simulink model "model"  (R2014b)
settings: Solver=ode4  StartTime=0.0  StopTime=10  FixedStep=0.01  RelTol=1e-3
values from neighbouring files (symbols this model uses):
  alp_trim = [0.0586239258484  0.0724982110928  0.103723100468; 0.0422368784565  0.0555720453493  0.0854543358165; 0.0309898683799  0.0444507527561  0.0743831948455]    [matlab.mat]    (also in plot_result.m = simOut.get('alp_trim')*r2d; plot_result_2.m = simOut.get('alp_trim')*r2d)
  dele_trim = [-0.00382132885472  -0.0381952981036  -0.0862584503139; 0.004502506619  -0.0421428537274  -0.104658611065; 0.0106660878134  -0.0496771115948  -0.12971922856]    [matlab.mat]
  delt_trim = [0.188785278717  0.195588305395  0.214097966619; 0.206526466279  0.211744859207  0.226730875318; 0.229775096744  0.233650878336  0.246767074549]    [matlab.mat]    (also in plot_result.m = simOut.get('delt_trim'); plot_result_2.m = simOut.get('delt_trim'))
undefined symbols (not defined in the file or in its folder): sigbuilder_block
libraries: aerolibconvert2 x9, LPVBlockLibrary x1, aerolibactuator x1
settings Model: Creator=jihoo  LastModifiedBy=Jihoon Lee

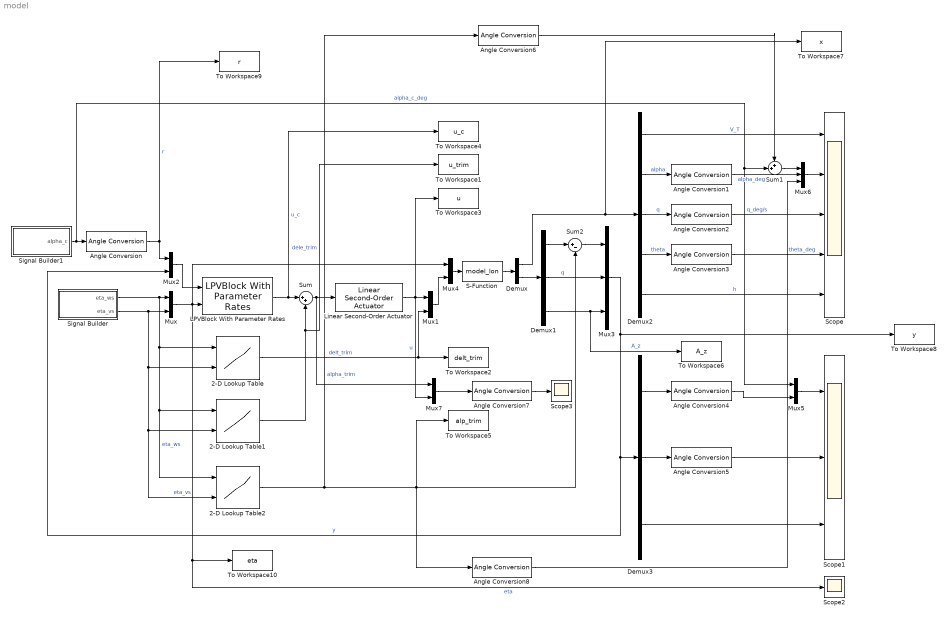
== system model ==
  2-D Lookup Table : Lookup_n-D  BreakpointsForDimension1=[0:0.5:1]  BreakpointsForDimension2=[0:0.5:1]  Table=delt_trim  InternalRulePriority=Speed  RndMeth=Simplest  InputSameDT=on
  2-D Lookup Table1 : Lookup_n-D  BreakpointsForDimension1=[0:0.5:1]  BreakpointsForDimension2=[0:0.5:1]  Table=dele_trim  InternalRulePriority=Speed  RndMeth=Simplest  InputSameDT=on
  2-D Lookup Table2 : Lookup_n-D  BreakpointsForDimension1=[0:0.5:1]  BreakpointsForDimension2=[0:0.5:1]  Table=alp_trim  InternalRulePriority=Speed  RndMeth=Simplest  InputSameDT=on
  Angle Conversion : aerolibconvert2/Angle Conversion  IU=deg  OU=rad
  Angle Conversion{1..8} (8 alike) : aerolibconvert2/Angle Conversion  IU=rad  OU=deg
  Demux : Demux  Outputs=[5 3]
  Demux1 : Demux  Outputs=[1 1 1]
  Demux2 : Demux  Outputs=5
  Demux3 : Demux  Outputs=3
  LPVBlock With Parameter Rates : LPVBlockLibrary/LPVBlock With Parameter Rates  sys=Knr  plist={'eta1';'eta2'}  x0=zeros(7,1)  ratetc={'eta1',0.5;'eta2',0.5}
  Linear Second-Order Actuator : aerolibactuator/Linear Second-Order Actuator  wn_fin=105  z_fin=0.6  fin_act_0=dele_trim(1,2)  fin_act_vel=0
  Mux : Mux  Inputs=2
  Mux1 : Mux  Inputs=2
  Mux2 : Mux  Inputs=[1 3]
  Mux3 : Mux  Inputs=[1 1 1]
  Mux4 : Mux  Inputs=[2 2]
  Mux5 : Mux  Inputs=2
  Mux6 : Mux  Inputs=[1 1 1]
  Mux7 : Mux  Inputs=[1 1]
  S-Function : S-Function  FunctionName=model_lon  EnableBusSupport=off
  Scope : Scope  NumInputPorts=5
      settings: YMin=16~2~-15~-10~294  YMax=24~5.5~10~15~308
  Scope1 : Scope  NumInputPorts=3
      settings: YMin=-5~-5~-5  YMax=5~5~5
  Scope2 : Scope
      settings: SaveName=ScopeData2
  Scope3 : Scope
      settings: ShowLegends=on  YMin=-8  YMax=1  SaveName=ScopeData3
  Signal Builder : Subsystem  Tag=STV Subsys  LoadFcn=sigbuilder_block('load',[0 -216 1861.5 1017 ]);  StartFcn=sigbuilder_block('start');  StopFcn=sigbuilder_block('stop');  ClipboardFcn=sigbuilder_block('clipboard');  mask(Sigbuilder block){}
      mask help: Simulink:masks:SigbuilderBlock_MD
      mask init:
      | if ~strcmp(get_param(bdroot(gcbh),'SimulationStatus'),'stopped') tuvar = sigbuilder_block('maskInit'); end
      settings: CopyFcn=sigbuilder_block('copy');  DeleteFcn=sigbuilder_block('delete');  ModelCloseFcn=sigbuilder_block('modelClose');  PreSaveFcn=sigbuilder_block('preSave');  PauseFcn=sigbuilder_block('pause');  ContinueFcn=sigbuilder_block('continue');  NameChangeFcn=sigbuilder_block('namechange');  OpenFcn=sigbuilder_block('open',[437.6 199.2 550.4 400 ]);  CloseFcn=sigbuilder_block('close');
      mask Display: plot(0, 0, 100, 100,[2, 2, 32, 32, 2], [68, 8, 8, 68, 68],[32, 2], [38, 38], [32, 19, 2],[53, 60, 44], [32, 17, 17, 2],[16, 16, 31, 31]);txt = getActiveGroup(gcbh);text(2, 100, txt,'verticalAlignment', 'top');
  Signal Builder1 : Subsystem  Tag=STV Subsys  LoadFcn=sigbuilder_block('load');  StartFcn=sigbuilder_block('start');  StopFcn=sigbuilder_block('stop');  ClipboardFcn=sigbuilder_block('clipboard');  mask(Sigbuilder block){}
      mask help: Simulink:masks:SigbuilderBlock_MD
      mask init:
      | if ~strcmp(get_param(bdroot(gcbh),'SimulationStatus'),'stopped') tuvar = sigbuilder_block('maskInit'); end
      settings: CopyFcn=sigbuilder_block('copy');  DeleteFcn=sigbuilder_block('delete');  ModelCloseFcn=sigbuilder_block('modelClose');  PreSaveFcn=sigbuilder_block('preSave');  PauseFcn=sigbuilder_block('pause');  ContinueFcn=sigbuilder_block('continue');  NameChangeFcn=sigbuilder_block('namechange');  OpenFcn=sigbuilder_block('open',[437.6 199.2 550.4 400 ]);  CloseFcn=sigbuilder_block('close');
      mask Display: plot(0, 0, 100, 100,[2, 2, 32, 32, 2], [68, 8, 8, 68, 68],[32, 2], [38, 38], [32, 19, 2],[53, 60, 44], [32, 17, 17, 2],[16, 16, 31, 31]);txt = getActiveGroup(gcbh);text(2, 100, txt,'verticalAlignment', 'top');
  Sum : Sum  Inputs=|++
  Sum1 : Sum  Inputs=++|
  Sum2 : Sum  Inputs=|+-
  To Workspace1 : ToWorkspace  VariableName=u_trim  SampleTime=-1
      settings: Save2DSignal=2-D array (concatenate along first dimension)
  To Workspace10 : ToWorkspace  VariableName=eta  SampleTime=-1
      settings: Save2DSignal=2-D array (concatenate along first dimension)
  To Workspace2 : ToWorkspace  VariableName=delt_trim  SampleTime=-1
      settings: Save2DSignal=2-D array (concatenate along first dimension)
  To Workspace3 : ToWorkspace  VariableName=u  SampleTime=-1
      settings: Save2DSignal=2-D array (concatenate along first dimension)
  To Workspace4 : ToWorkspace  VariableName=u_c  SampleTime=-1
      settings: Save2DSignal=2-D array (concatenate along first dimension)
  To Workspace5 : ToWorkspace  VariableName=alp_trim  SampleTime=-1
      settings: Save2DSignal=2-D array (concatenate along first dimension)
  To Workspace6 : ToWorkspace  VariableName=A_z  SampleTime=-1
      settings: Save2DSignal=2-D array (concatenate along first dimension)
  To Workspace7 : ToWorkspace  VariableName=x  SampleTime=-1
      settings: Save2DSignal=2-D array (concatenate along first dimension)
  To Workspace8 : ToWorkspace  VariableName=y  SampleTime=-1
      settings: Save2DSignal=2-D array (concatenate along first dimension)
  To Workspace9 : ToWorkspace  VariableName=r  SampleTime=-1
      settings: Save2DSignal=2-D array (concatenate along first dimension)
  wires:
  Signal Builder/1(eta_ws) -> 2-D Lookup Table2/1, 2-D Lookup Table1/1, 2-D Lookup Table/1, Mux/1  "eta_ws"
  Signal Builder/2(eta_vs) -> 2-D Lookup Table2/2, 2-D Lookup Table1/2, 2-D Lookup Table/2, Mux/2  "eta_vs"
  Mux/1 -> Mux4/1, To Workspace10/1, Scope2/1, LPVBlock With Parameter Rates/2  "eta"
  S-Function/1 -> Demux/1
  Mux2/1 -> LPVBlock With Parameter Rates/1
  LPVBlock With Parameter Rates/1 -> To Workspace4/1, Sum/1  "u_c"
  2-D Lookup Table/1 -> To Workspace2/1, Mux1/2  "delt_trim"
  2-D Lookup Table1/1 -> To Workspace1/1, Sum/2  "dele_trim"
  2-D Lookup Table2/1 -> Angle Conversion6/1, Angle Conversion8/1, To Workspace5/1, Sum2/2  "alpha_trim"
  Demux/2 -> Demux1/1
  Demux/1 -> To Workspace7/1, Demux2/1
  Demux1/1 -> Sum2/1
  Sum2/1 -> Mux3/1
  Demux1/2 -> Mux3/2  "q"
  Demux1/3 -> To Workspace6/1, Mux3/3  "A_z"
  Mux3/1 -> Demux3/1, Mux2/2, To Workspace8/1  "y"
  Angle Conversion/1 -> Mux2/1, To Workspace9/1  "r"
  Sum/1 -> Linear Second-Order Actuator/1, Mux7/1
  Linear Second-Order Actuator/1 -> Mux7/2, To Workspace3/1, Mux1/1  "u"
  Mux4/1 -> S-Function/1
  Mux1/1 -> Mux4/2
  Demux3/1 -> Angle Conversion4/1
  Demux3/2 -> Angle Conversion5/1
  Demux3/3 -> Scope1/3
  Demux2/1 -> Scope/1  "V_T"
  Demux2/2 -> Angle Conversion1/1  "alpha"
  Demux2/3 -> Angle Conversion2/1  "q"
  Demux2/4 -> Angle Conversion3/1  "theta"
  Demux2/5 -> Scope/5  "h"
  Angle Conversion2/1 -> Scope/3  "q_deg/s"
  Angle Conversion3/1 -> Scope/4  "theta_deg"
  Angle Conversion5/1 -> Scope1/2
  Mux5/1 -> Scope1/1
  Angle Conversion4/1 -> Mux5/2
  Signal Builder1/1(alpha_c) -> Sum1/2, Mux5/1, Angle Conversion/1  "alpha_c_deg"
  Mux6/1 -> Scope/2
  Angle Conversion1/1 -> Mux6/2  "alpha_deg"
  Sum1/1 -> Mux6/1
  Angle Conversion6/1 -> Sum1/1
  Mux7/1 -> Angle Conversion7/1
  Angle Conversion7/1 -> Scope3/1
  Angle Conversion8/1 -> Mux6/3

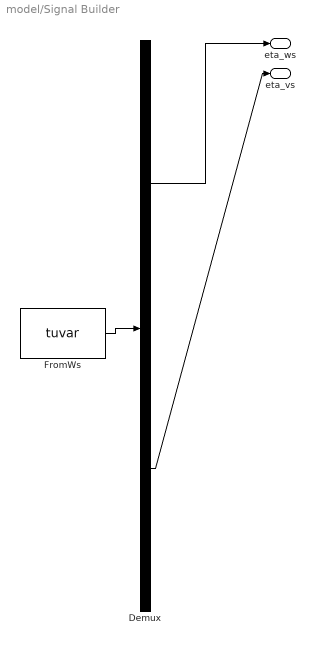
== system model/Signal Builder ==
  Demux : Demux  Tag=STV Demux  Outputs=2
  FromWs : FromWorkspace  Tag=STV FromWs  VariableName=tuvar  SampleTime=0
      SigBuilderData=|
      | common.afterFinalStr = 'Extrapolate'
      | common.sampleTime = 0
      | dataSet.timeRange = [0 20]
      | dataSet.name = 'eta'
      | sbobj.Groups.Name = 'eta'
      | sbobj.Groups.Signals(1).Name = 'eta_ws'
      | sbobj.Groups.Signals(1).XData = [0 2 3 5 20]
      | sbobj.Groups.Signals(1).YData = [0 1 1 0 0]
      | sbobj.Groups.Signals(2).Name = 'eta_vs'
      | sbobj.Groups.Signals(2).XData = [0 1 3 4 6 20]
      | sbobj.Groups.Signals(2).YData = [0.5 0 1 1 0 0]
      | sbobj.Groups.TimeRange = [0 20]
  eta_ws : Outport  Tag=STV Outport
  eta_vs : Outport  Tag=STV Outport  Port=2
  wires:
  Demux/1 -> eta_ws/1
  FromWs/1 -> Demux/1
  Demux/2 -> eta_vs/1

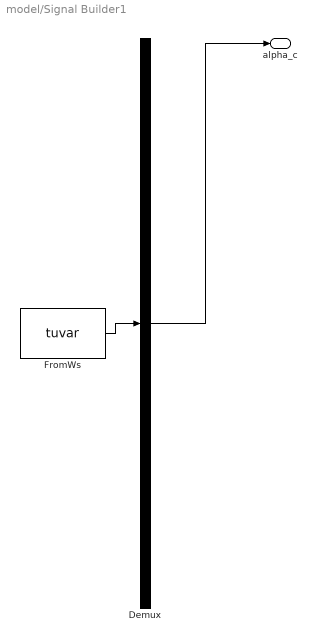
== system model/Signal Builder1 ==
  Demux : Demux  Tag=STV Demux  Outputs=1
  FromWs : FromWorkspace  Tag=STV FromWs  VariableName=tuvar  SampleTime=0
      SigBuilderData=|
      | common.afterFinalStr = 'Extrapolate'
      | common.sampleTime = 0
      | dataSet.timeRange = [0 20]
      | dataSet.name = 'command'
      | sbobj.Groups.Name = 'command'
      | sbobj.Groups.Signals.Name = 'alpha_c'
      | sbobj.Groups.Signals.XData = [0 2.5 2.5 20]
      | sbobj.Groups.Signals.YData = [1 1 0 0]
      | sbobj.Groups.TimeRange = [0 20]
  alpha_c : Outport  Tag=STV Outport
  wires:
  Demux/1 -> alpha_c/1
  FromWs/1 -> Demux/1
